simulink model "model"  (R2025b)
settings: Solver=ode4  StartTime=0.0  StopTime=200  FixedStep=0.005  RelTol=1e-3
InitFcn:
  | clear xlog terms ulog cmdlog phaselog tvclog
  | run(fullfile(fileparts(get_param(bdroot, 'FileName')), 'rocket_init.m'));
StopFcn:
  | if exist('show_replay', 'var') && show_replay && exist('xlog', 'var')
  |     bsim.rocket.after_run(bdroot, xlog, terms, Prk, 'U', ulog);
  | end
values from neighbouring files (symbols this model uses):
  Prk = bsim.rocket.pack(S)    [rocket_init.m]
  Ptvc = bsim.tvc.pack(bsim.tvc.params('ember'))    [rocket_init.m]
undefined symbols (not defined in the file or in its folder): act, x0
libraries: simulink x2
settings Model: Creator=lukascampbell  LastModifiedBy=lukascampbell
settings DataIOCC: ReturnWorkspaceOutputs=off
settings SFSimCC: SimCustomHeaderCode="#include \"bsim_c.h\""  SimUserIncludeDirs=/Users/lukascampbell/Documents/GitHub/6dof-uav-sim/matlab/bridge  SimUserLibraries=/Users/lukascampbell/Documents/GitHub/6dof-uav-sim/matlab/bin/libbsim_c.dylib  DefaultCustomCodeDeterministicFunctions=All

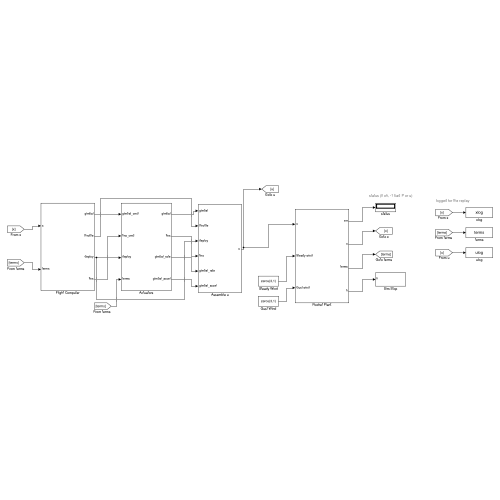
[thumbnail: Simulink's stored preview of the top-level diagram]
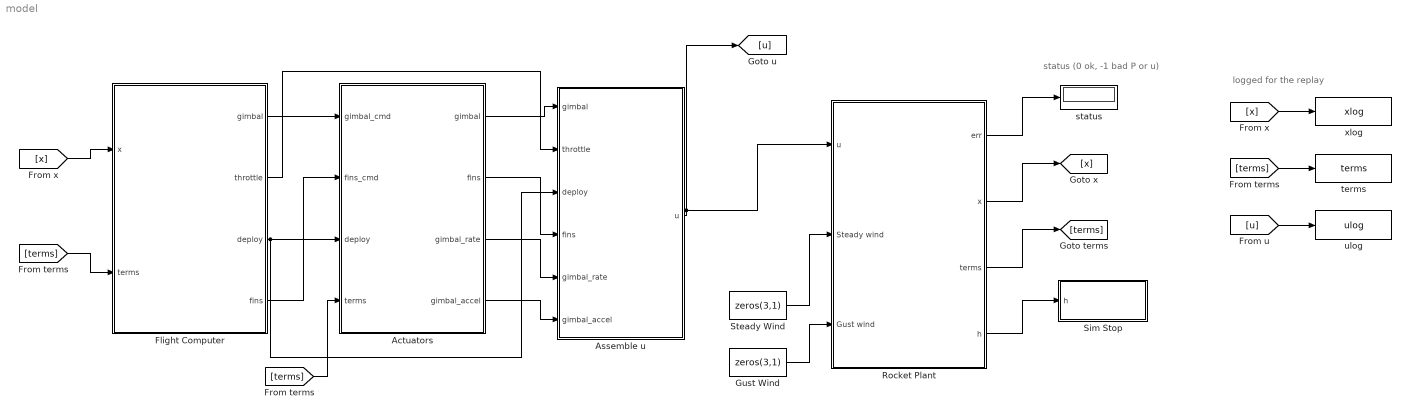
== system model ==
  note: status (0 ok, -1 bad P or u)
  note: logged for the replay
  Actuators : Subsystem
  Assemble u : Subsystem
  Flight Computer : Subsystem
  Gust Wind : Constant  Value=zeros(3,1)
  Rocket Plant : Subsystem
  Sim Stop : Subsystem
  Steady Wind : Constant  Value=zeros(3,1)
  status : Display
  terms : ToWorkspace  VariableName=terms  SaveFormat=Timeseries  SampleTime=-1
  ulog : ToWorkspace  VariableName=ulog  SaveFormat=Timeseries  SampleTime=-1
  xlog : ToWorkspace  VariableName=xlog  SaveFormat=Timeseries  SampleTime=-1
  wires:
  [x] -> Flight Computer/1(x)
  [terms] -> Flight Computer/2(terms)
  Flight Computer/1(gimbal) -> Actuators/1(gimbal_cmd)
  Flight Computer/4(fins) -> Actuators/2(fins_cmd)
  Flight Computer/3(deploy) -> Actuators/3(deploy), Assemble u/3(deploy)
  Actuators/1(gimbal) -> Assemble u/1(gimbal)
  Flight Computer/2(throttle) -> Assemble u/2(throttle)
  Actuators/2(fins) -> Assemble u/4(fins)
  Assemble u/1("u ") -> Rocket Plant/1(u), [u]
  Steady Wind/1 -> Rocket Plant/2(Steady wind)
  Gust Wind/1 -> Rocket Plant/3(Gust wind)
  Rocket Plant/1(err) -> status/1
  Rocket Plant/2(x) -> [x]
  Rocket Plant/3(terms) -> [terms]
  Rocket Plant/4(h) -> Sim Stop/1(h)
  [x] -> xlog/1
  [terms] -> terms/1
  [u] -> ulog/1
  Actuators/3(gimbal_rate) -> Assemble u/5(gimbal_rate)
  Actuators/4(gimbal_accel) -> Assemble u/6(gimbal_accel)
  [terms] -> Actuators/4(terms)

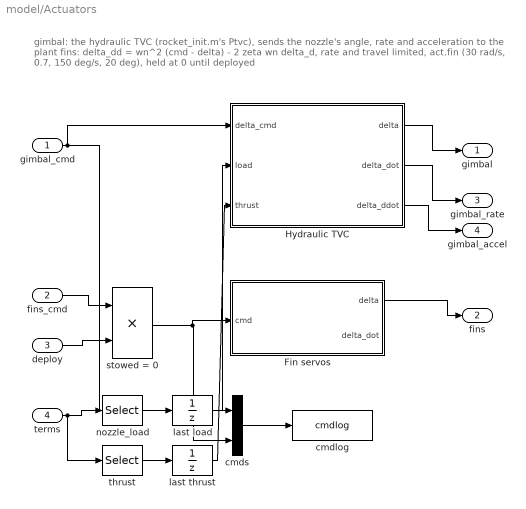
== system model/Actuators ==
  note: gimbal: the hydraulic TVC (rocket_init.m's Ptvc), sends the nozzle's angle, rate and acceleration to the plant
      | fins: delta_dd = wn^2 (cmd - delta) - 2 zeta wn delta_d, rate and travel limited, act.fin (30 rad/s, 0.7, 150 deg/s, 20 deg), held at 0 until deployed
  gimbal_cmd : Inport
  fins_cmd : Inport  Port=2
  deploy : Inport  Port=3
  terms : Inport  Port=4
  Fin servos : Subsystem
  Hydraulic TVC : Subsystem  TreatAsAtomicUnit=on  SystemSampleTime=0.005
  cmdlog : ToWorkspace  VariableName=cmdlog  SaveFormat=Timeseries  SampleTime=-1
  cmds : Concatenate
  last load : UnitDelay  InitialCondition=zeros(2,1)  SampleTime=0.005  HasFrameUpgradeWarning=on
  last thrust : UnitDelay  SampleTime=0.005  HasFrameUpgradeWarning=on
  nozzle_load : Selector  InputPortWidth=41  IndexOptions=Index vector (dialog)  Indices=[40 41]  OutputSizes=1
  stowed = 0 : Product
  thrust : Selector  InputPortWidth=41  IndexOptions=Index vector (dialog)  Indices=5  OutputSizes=1
  gimbal : Outport
  fins : Outport  Port=2
  gimbal_rate : Outport  Port=3
  gimbal_accel : Outport  Port=4
  wires:
  gimbal_cmd/1 -> cmds/1, Hydraulic TVC/1(delta_cmd)
  fins_cmd/1 -> stowed = 0/1
  deploy/1 -> stowed = 0/2
  stowed = 0/1 -> Fin servos/1(cmd), cmds/2
  cmds/1 -> cmdlog/1
  Fin servos/1(delta) -> fins/1
  terms/1 -> nozzle_load/1, thrust/1
  nozzle_load/1 -> last load/1
  thrust/1 -> last thrust/1
  last load/1 -> Hydraulic TVC/2(load)
  last thrust/1 -> Hydraulic TVC/3(thrust)
  Hydraulic TVC/1("delta ") -> gimbal/1
  Hydraulic TVC/2(delta_dot) -> gimbal_rate/1
  Hydraulic TVC/3(delta_ddot) -> gimbal_accel/1

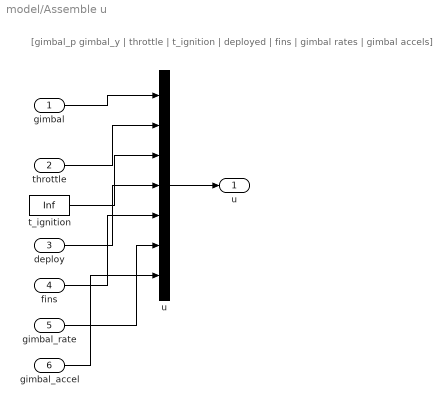
== system model/Assemble u ==
  note: [gimbal_p gimbal_y | throttle | t_ignition | deployed | fins | gimbal rates | gimbal accels]
  gimbal : Inport
  throttle : Inport  Port=2
  deploy : Inport  Port=3
  fins : Inport  Port=4
  gimbal_rate : Inport  Port=5
  gimbal_accel : Inport  Port=6
  t_ignition : Constant  Value=Inf
  u : Concatenate  NumInputs=7
  "u " : Outport
  wires:
  gimbal/1 -> u/1
  throttle/1 -> u/2
  t_ignition/1 -> u/3
  deploy/1 -> u/4
  fins/1 -> u/5
  u/1 -> "u "/1
  gimbal_rate/1 -> u/6
  gimbal_accel/1 -> u/7

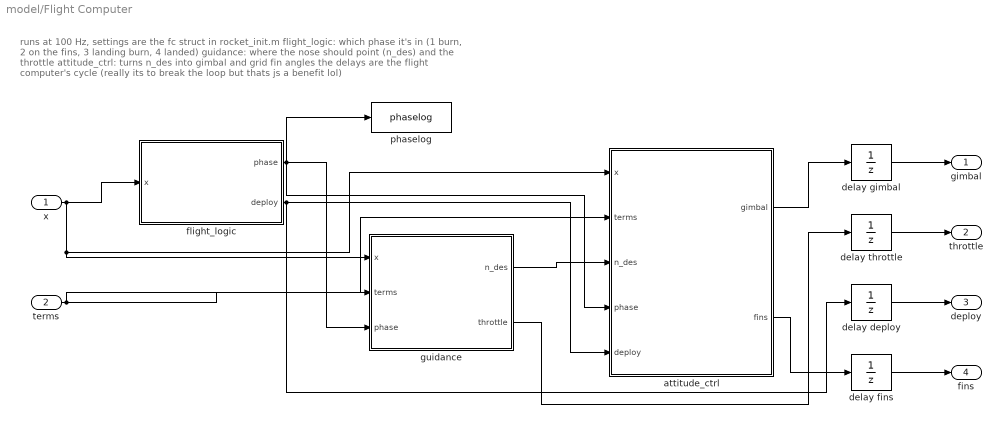
== system model/Flight Computer ==
  note: runs at 100 Hz, settings are the fc struct in rocket_init.m
      | flight_logic: which phase it's in (1 burn, 2 on the fins, 3 landing burn, 4 landed)
      | guidance: where the nose should point (n_des) and the throttle
      | attitude_ctrl: turns n_des into gimbal and grid fin angles
      | the delays are the flight computer's cycle (really its to break the loop but thats js a benefit lol)
  x : Inport
  terms : Inport  Port=2
  attitude_ctrl : MATLAB Function  TreatAsAtomicUnit=on  SystemSampleTime=0.01
  delay deploy : UnitDelay  SampleTime=0.01  HasFrameUpgradeWarning=on
  delay fins : UnitDelay  InitialCondition=zeros(4,1)  SampleTime=0.01  HasFrameUpgradeWarning=on
  delay gimbal : UnitDelay  InitialCondition=zeros(2,1)  SampleTime=0.01  HasFrameUpgradeWarning=on
  delay throttle : UnitDelay  SampleTime=0.01  HasFrameUpgradeWarning=on
  flight_logic : MATLAB Function  TreatAsAtomicUnit=on  SystemSampleTime=0.01
  guidance : MATLAB Function  TreatAsAtomicUnit=on  SystemSampleTime=0.01
  phaselog : ToWorkspace  VariableName=phaselog  SaveFormat=Timeseries  SampleTime=-1
  gimbal : Outport
  throttle : Outport  Port=2
  deploy : Outport  Port=3
  fins : Outport  Port=4
  wires:
  delay gimbal/1 -> gimbal/1
  delay throttle/1 -> throttle/1
  delay deploy/1 -> deploy/1
  delay fins/1 -> fins/1
  x/1 -> guidance/1(x), attitude_ctrl/1(x), flight_logic/1(x)
  terms/1 -> guidance/2(terms), attitude_ctrl/2(terms)
  flight_logic/1(phase) -> guidance/3(phase), attitude_ctrl/4(phase), phaselog/1
  guidance/1(n_des) -> attitude_ctrl/3(n_des)
  flight_logic/2(deploy) -> attitude_ctrl/5(deploy), delay deploy/1
  attitude_ctrl/1(gimbal) -> delay gimbal/1
  guidance/2(throttle) -> delay throttle/1
  attitude_ctrl/2(fins) -> delay fins/1

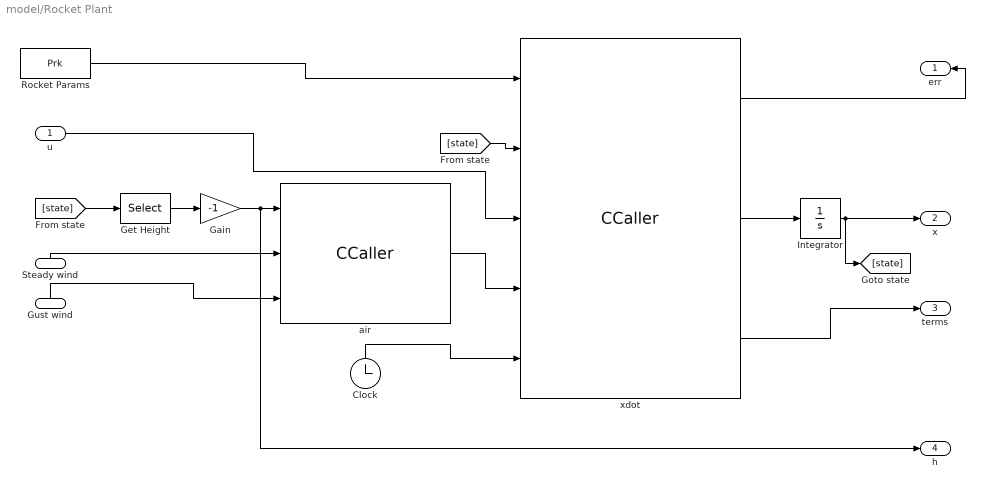
== system model/Rocket Plant ==
  u : Inport
  Steady wind : Inport  Port=2
  Gust wind : Inport  Port=3
  Clock : Clock
  Gain : Gain  Gain=-1
  Get Height : Selector  InputPortWidth=14  IndexOptions=Index vector (dialog)  Indices=3  OutputSizes=1
  Integrator : Integrator  InitialCondition=x0
  Rocket Params : Constant  Value=Prk
  air : CCaller  FunctionName=bsim_isa_rocket_air  PortSpecificationStruct="%)30     .    & <   8    (     @         %    \"     0    !     0         %  0 \"0    $    _    07)G3F%M90  4&]R=$YA;64 4V-O<&4     26YD97@     5'EP90      4VEZ90      27-';&]B86P   X    P    !@    @    $          4    (     0    $    !         !   0!H    #@   #     &    \"     0         !0    @    !     0    $         $  ! &@    .    .     8    (    !          %    \"     $    %     0         0   ...(+2058 chars)"
  xdot : CCaller  FunctionName=bsim_rocket_xdot  PortSpecificationStruct="%)30     .    Z!    8    (     @         %    \"     H    !     0         %  0 \"0    $    _    07)G3F%M90  4&]R=$YA;64 4V-O<&4     26YD97@     5'EP90      4VEZ90      27-';&]B86P   X    P    !@    @    $          4    (     0    ,    !         !   P!O=70 #@   #     &    \"     0         !0    @    !     P    $         $  # &]U=  .    .     8    (    !          %    \"     $    &     0         0   ...(+5457 chars)"
  err : Outport
  x : Outport  Port=2
  terms : Outport  Port=3
  h : Outport  Port=4
  wires:
  Rocket Params/1 -> xdot/1
  [state] -> xdot/2
  u/1 -> xdot/3
  air/1 -> xdot/4
  Clock/1 -> xdot/5
  Steady wind/1 -> air/2
  Gust wind/1 -> air/3
  xdot/2 -> Integrator/1
  Integrator/1 -> x/1, [state]
  [state] -> Get Height/1
  Get Height/1 -> Gain/1
  Gain/1 -> air/1, h/1
  xdot/1 -> err/1
  xdot/3 -> terms/1

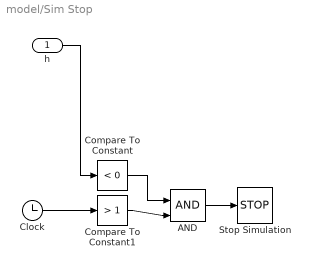
== system model/Sim Stop ==
  h : Inport
  AND : Logic  IconShape=distinctive  AllPortsSameDT=off  OutDataTypeStr=boolean
  Clock : Clock
  Compare To Constant : simulink/Logic and Bit Operations/Compare To Constant  relop=<  const=0  OutDataTypeStr=boolean
  Compare To Constant1 : simulink/Logic and Bit Operations/Compare To Constant  relop=>  const=1  OutDataTypeStr=boolean
  Stop Simulation : Stop
  wires:
  AND/1 -> Stop Simulation/1
  Compare To Constant/1 -> AND/1
  h/1 -> Compare To Constant/1
  Compare To Constant1/1 -> AND/2
  Clock/1 -> Compare To Constant1/1

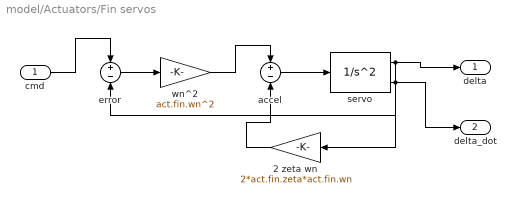
== system model/Actuators/Fin servos ==
  cmd : Inport
  2 zeta wn : Gain  Gain=2*act.fin.zeta*act.fin.wn
  accel : Sum  Inputs=+-
  error : Sum  Inputs=+-
  servo : SecondOrderIntegrator  ICX=0  LimitX=on  UpperLimitX=act.fin.pos_max  LowerLimitX=-act.fin.pos_max  ICDXDT=0  LimitDXDT=on  UpperLimitDXDT=act.fin.rate_max  LowerLimitDXDT=-act.fin.rate_max  ReinitDXDTwhenXreachesSaturation=on
  wn^2 : Gain  Gain=act.fin.wn^2
  delta : Outport
  delta_dot : Outport  Port=2
  wires:
  cmd/1 -> error/1
  error/1 -> wn^2/1
  wn^2/1 -> accel/1
  accel/1 -> servo/1
  servo/1 -> delta/1, error/2
  servo/2 -> delta_dot/1, 2 zeta wn/1
  2 zeta wn/1 -> accel/2

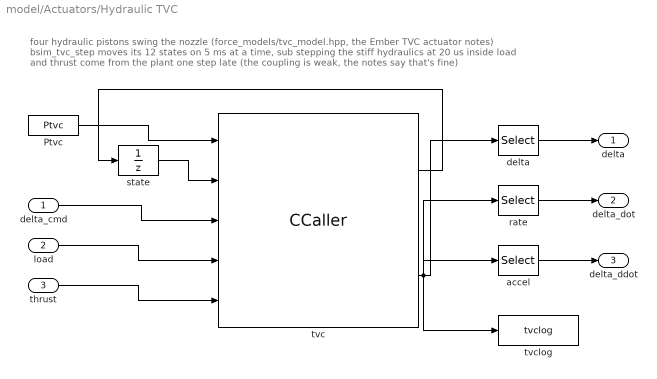
== system model/Actuators/Hydraulic TVC ==
  note: four hydraulic pistons swing the nozzle (force_models/tvc_model.hpp, the Ember TVC actuator notes)
      | bsim_tvc_step moves its 12 states on 5 ms at a time, sub stepping the stiff hydraulics at 20 us inside
      | load and thrust come from the plant one step late (the coupling is weak, the notes say that's fine)
  delta_cmd : Inport
  load : Inport  Port=2
  thrust : Inport  Port=3
  Ptvc : Constant  Value=Ptvc
  accel : Selector  InputPortWidth=18  IndexOptions=Index vector (dialog)  Indices=[5 6]  OutputSizes=1
  delta : Selector  InputPortWidth=18  IndexOptions=Index vector (dialog)  Indices=[1 2]  OutputSizes=1
  rate : Selector  InputPortWidth=18  IndexOptions=Index vector (dialog)  Indices=[3 4]  OutputSizes=1
  state : UnitDelay  InitialCondition=zeros(12,1)  SampleTime=0.005  HasFrameUpgradeWarning=on
  tvc : CCaller  FunctionName=bsim_tvc_step  PortSpecificationStruct="%)30     .    L T   8    (     @         %    \"     @    !     0         %  0 \"0    $    _    07)G3F%M90  4&]R=$YA;64 4V-O<&4     26YD97@     5'EP90      4VEZ90      27-';&]B86P   X    P    !@    @    $          4    (     0    $    !         !   0!0    #@   #     &    \"     0         !0    @    !     0    $         $  ! %     .    .     8    (    !          %    \"     $    %     0         0   ...(+4351 chars)"
  tvclog : ToWorkspace  VariableName=tvclog  SaveFormat=Timeseries  SampleTime=-1
  "delta " : Outport
  delta_dot : Outport  Port=2
  delta_ddot : Outport  Port=3
  wires:
  Ptvc/1 -> tvc/1
  state/1 -> tvc/2
  delta_cmd/1 -> tvc/3
  load/1 -> tvc/4
  thrust/1 -> tvc/5
  tvc/1 -> state/1
  tvc/2 -> delta/1, rate/1, accel/1, tvclog/1
  delta/1 -> "delta "/1
  rate/1 -> delta_dot/1
  accel/1 -> delta_ddot/1

== matlab function model/Flight Computer/guidance ==
  data: x input; n_des output size=[3,1]; terms input; phase input; throttle output size=[1,1]; fc parameter
function [n_des, throttle] = guidance(x, terms, phase, fc)
% where the nose should point (n_des, a unit vector in NED, or zeros for "just damp") and
% the throttle, for each phase of the flight (see flight_logic)
r = x(1:3);                 % position, NED [m]
v = x(4:6);                 % velocity, NED [m/s]
h = -r(3);
m = x(14);
qbar = terms(9);            % dynamic pressure [Pa]
alpha_t = terms(10);        % angle between the nose and the airflow [rad]
F_aero = terms(17:19);      % aero force, body [N]
g = terms(25);              % gravity (down) [m/s^2]
R = dcm(x(7:10));           % body -> NED
v_air = R * terms(32:34);   % velocity relative to the air, NED

n_des = zeros(3, 1);
throttle = 0;
switch phase
    case 1
        % burn: straight up, full throttle
        n_des = [0; 0; -1];
        throttle = 1;

    case 2
        % falling on the fins: tail into the airflow, leaning a little to steer at the target
        if alpha_t > deg2rad(150) && qbar > 50 && norm(v_air) > 1
            into_air = -v_air / norm(v_air);           % straight into the air coming up at it
            a_h = fc.kp_fin * (fc.target - r(1:2)) - fc.kd_fin * v(1:2);
            % falling tail first, leaning the nose one way pushes the rocket the other
            % (fc.k_tilt < 0, measured from the model), and the fins can only hold a few degrees
            lean = a_h / (fc.k_tilt * qbar);
            if norm(lean) > fc.lean_max
                lean = lean * fc.lean_max / norm(lean);
            end
            n = into_air + [lean; 0];
            n_des = n / norm(n);
        end

    case 3
        % landing burn: thrust along the nose, so point it along the acceleration we want
        v_down = v(3);
        % how fast to be falling here: slowing at a_land on the way down, reaching v_touch at
        % h_flare, then coming down the last bit at v_touch
        v_ref = sqrt(fc.v_touch^2 + 2 * fc.a_land * max(h - fc.h_flare, 0));
        a_up = fc.a_land * (h > fc.h_flare) + fc.kv * (v_down - v_ref);   % follow it (feedforward + correction)
        % sideways: arrive over the target with no sideways speed, at the same time as touchdown
        % (t_go = how long the rest of the burn takes), a = 6 dr / t_go^2 - 4 v / t_go
        % in the last couple of seconds it just stops sliding and stands up (touching down upright
        % and slow matters more than the last few metres)
        t_go = v_down / fc.a_land;
        if t_go > fc.t_final
            a_h = 6 * (fc.target - r(1:2)) / t_go^2 - 4 * v(1:2) / t_go;
        else
            a_h = -v(1:2) / fc.tau_final;
        end
        a_h_max = fc.tilt_max * (g + a_up);
        if norm(a_h) > a_h_max
            a_h = a_h * a_h_max / max(norm(a_h), 1e-9);
        end
        a_want = [a_h; -a_up];                         % NED
        a_thrust = a_want - [0; 0; g] - R * F_aero / m; % what the engine has to supply
        T_need = m * norm(a_thrust);
        n_des = a_thrust / max(norm(a_thrust), 1e-9);
        if n_des(3) > -0.5                             % never more than 60 deg off vertical
            n_des = [0; 0; -1];
        end
        throttle = (T_need + fc.p_Ae) / fc.T_vac;
        throttle = min(1, max(fc.throttle_min + 0.01, throttle));

    otherwise
        % landed
        n_des = [0; 0; -1];
        throttle = 0;
end
end

function R = dcm(q)
% body -> NED rotation from the [e0 e1 e2 e3] quaternion
q = q / norm(q);
e0 = q(1); e1 = q(2); e2 = q(3); e3 = q(4);
R = [e1^2+e0^2-e2^2-e3^2, 2*(e1*e2-e3*e0),     2*(e1*e3+e2*e0);
     2*(e1*e2+e3*e0),     e2^2+e0^2-e1^2-e3^2, 2*(e2*e3-e1*e0);
     2*(e1*e3-e2*e0),     2*(e2*e3+e1*e0),     e3^2+e0^2-e1^2-e2^2];
end

== matlab function model/Flight Computer/flight_logic ==
  data: x input; phase output size=[1,1]; deploy output size=[1,1]; fc parameter
function [phase, deploy] = flight_logic(x, fc)
% which part of the flight it's in (holds its value between steps)
%   1 burn          engine on, gimbal keeps it straight
%   2 unpowered     MECO once the mass is down to fc.m_cut, fins out, falling on the fins
%   3 landing burn  relit once stopping fc.h_margin above the ground needs fc.a_ign of deceleration
%   4 landed        engine off
persistent ph
if isempty(ph)
    ph = 1;
end
h = -x(3);        % altitude [m] (x(3) is down)
v_down = x(6);    % [m/s], positive falling
m = x(14);        % mass [kg]

if ph == 1 && m <= fc.m_cut
    ph = 2;
elseif ph == 2 && v_down > 0 && h < fc.h_ign_max
    % constant deceleration needed to stop h_margin above the ground: v^2 / 2 d
    a_need = v_down^2 / (2 * max(h - fc.h_margin, 1));
    if a_need >= fc.a_ign
        ph = 3;
    end
elseif ph == 3 && h <= fc.h_cutoff
    ph = 4;
end
phase = ph;
deploy = double(ph >= 2);
end

== matlab function model/Flight Computer/attitude_ctrl ==
  data: x input; gimbal output size=[2,1]; terms input; n_des input; phase input; deploy input; fins output size=[4,1]; fc parameter
function [gimbal, fins] = attitude_ctrl(x, terms, n_des, phase, deploy, fc)
% turns "point the nose along n_des" into gimbal and grid fin angles
%   the gimbal does pitch/yaw whenever the engine is making thrust, the fins take whatever the
%   gimbal can't (and all of the roll) once they're out and there's air
gimbal = zeros(2, 1);
fins = zeros(4, 1);
Ix = terms(3);  It = terms(4);  x_cm = terms(2);
T = terms(5);  qbar = terms(9);  v_r = terms(32:34);
w = x(11:13);                       % body rates [p q r]
R = dcm(x(7:10));                   % body -> NED
nose = R(:, 1);

% pointing error as a small rotation in body axes (e(2) pitch, e(3) yaw); none to just damp
e = zeros(3, 1);
if norm(n_des) > 0.5
    e = R.' * cross(nose, n_des);
end

% PD on the pointing error, plus enough extra stiffness to beat the airframe's own
% (unstable) aero moment while it's going up nose first
wn = fc.wn;
Kp = It * wn^2;
if v_r(1) > 0
    Kp = Kp + fc.c_aero * qbar;
end
Kd = 2 * fc.zeta * wn * It;
M = [-fc.k_roll * Ix * w(1); Kp * e(2) - Kd * w(2); Kp * e(3) - Kd * w(3)];   % [N m]

% falling tail first the aero pulls the nose back into the airflow, so add the moment that holds it
% at n_des against that (without it, it only gets part way to a lean the guidance asks for)
if v_r(1) < 0 && norm(n_des) > 0.5 && norm(v_r) > 1
    into_air = -v_r / norm(v_r);                       % body axes
    hold_ = fc.c_aero * qbar * cross(into_air, R.' * n_des);
    M(2:3) = M(2:3) + hold_(2:3);
end

% gimbal: moment per rad is T (x_cm - x_G), measured from the model
if T > 100
    G = T * (x_cm - fc.x_G);
    gimbal = M(2:3) / G;
    gimbal = max(-fc.gimbal_max, min(fc.gimbal_max, gimbal));
    M(2:3) = M(2:3) - G * gimbal;   % what's left over for the fins
end

% fins: the mixer was measured tail first, they push the other way with air from the nose
if deploy > 0.5 && qbar > 50 && phase >= 2
    fins = -sign(v_r(1)) * (fc.Mfin * M) / qbar;
    fins = max(-fc.fin_max, min(fc.fin_max, fins));
end
end

function R = dcm(q)
q = q / norm(q);
e0 = q(1); e1 = q(2); e2 = q(3); e3 = q(4);
R = [e1^2+e0^2-e2^2-e3^2, 2*(e1*e2-e3*e0),     2*(e1*e3+e2*e0);
     2*(e1*e2+e3*e0),     e2^2+e0^2-e1^2-e3^2, 2*(e2*e3-e1*e0);
     2*(e1*e3-e2*e0),     2*(e2*e3+e1*e0),     e3^2+e0^2-e1^2-e2^2];
end
